simulink library "sfEngineTemperatureLibrary"  (R2025b)
settings: Solver=VariableStepAuto  StartTime=0.0  StopTime=10.0  RelTol=1e-3
settings Model: Creator=The MathWorks, Inc.  LastModifiedBy=The MathWorks, Inc.

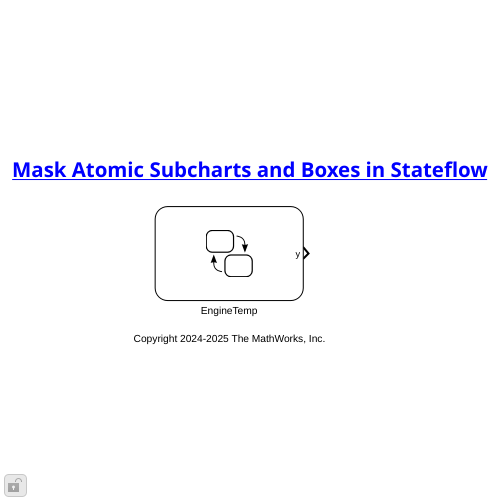
[thumbnail: Simulink's stored preview of the top-level diagram]
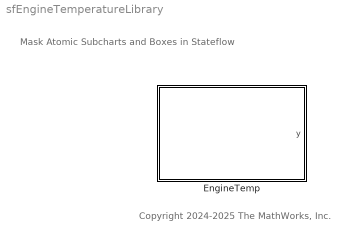
== system sfEngineTemperatureLibrary ==
  note: Copyright 2024-2025 The MathWorks, Inc.
  note: Mask Atomic Subcharts and Boxes in Stateflow
  EngineTemp : Stateflow chart  TreatAsAtomicUnit=on

== stateflow chart sfEngineTemperatureLibrary/EngineTemp ==
  state NORM
    y = 0;
  state WARN
    y = 1;
  state ALARM
    y = 2;
  (default) -> NORM
  NORM -> WARN : [temp > 190]
  WARN -> ALARM [order 2] : [temp > 225]
  WARN -> NORM [order 1] : [temp <= 190]
  ALARM -> WARN : [temp <= 225]
  data: y output double size=1; temp parameter
